simulink model "tuning_and_analysis"  (R2025b)
settings: Solver=ode45  StartTime=0.0  StopTime=0.1  RelTol=1e-6  AbsTol=1e-6
InitFcn:
  | init_pendulum
settings Model: Creator=Hp  LastModifiedBy=Hp

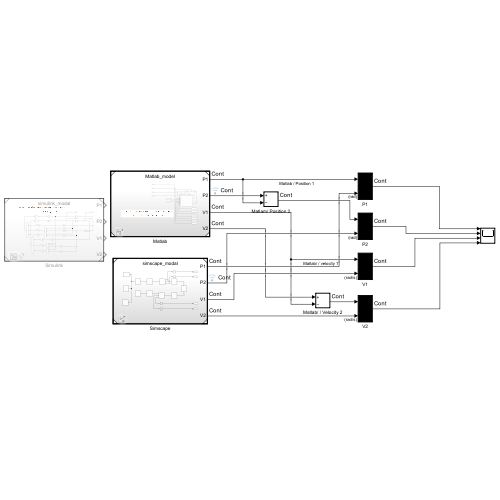
[thumbnail: Simulink's stored preview of the top-level diagram]
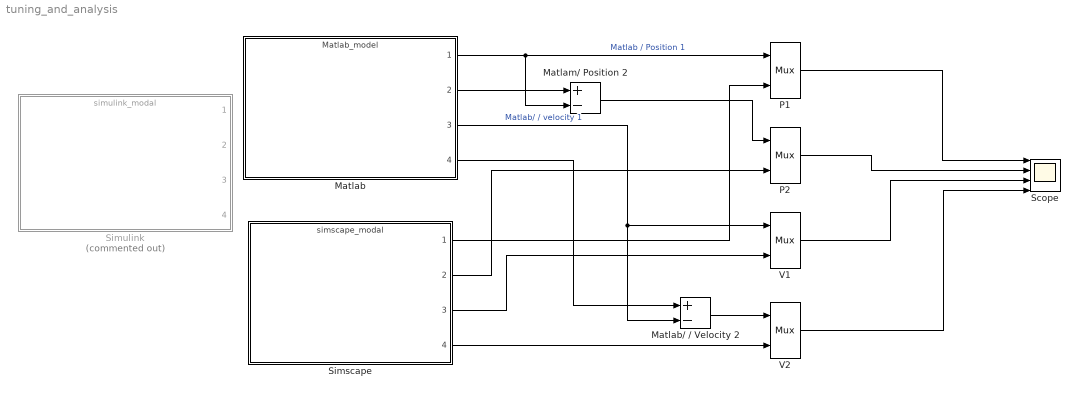
== system tuning_and_analysis ==
  Matlab : ModelReference  ModelNameDialog=Matlab_model.slx  SimulationMode=Normal  ModelReferenceVersion=1.11
  Matlab/ / Velocity 2 : Sum  Inputs=+-
  Matlam/ Position 2 : Sum  Inputs=+-
  P1 : Mux  Inputs=2
  P2 : Mux  Inputs=2
  Scope : Scope  NumInputPorts=4
      settings: ActiveDisplayYMinimum=-0.80264814806705076  ActiveDisplayYMaximum=-0.58955602599034473
  Simscape : ModelReference  ModelNameDialog=simscape_modal.slx  SimulationMode=Normal  ModelReferenceVersion=1.9
  Simulink : ModelReference  Commented=on  ModelNameDialog=simulink_modal.slx  SimulationMode=Normal  ModelReferenceVersion=1.5
  V1 : Mux  Inputs=2
  V2 : Mux  Inputs=2
  wires:
  P1/1 -> Scope/1
  P2/1 -> Scope/2
  Matlab/1 -> P1/1, Matlam/ Position 2/2  "Matlab / Position 1"
  Simscape/1 -> P1/2
  Simscape/2 -> P2/2
  Matlab/3 -> Matlab/ / Velocity 2/2, V1/1  "Matlab/ / velocity 1"
  Simscape/3 -> V1/2
  Simscape/4 -> V2/2
  Matlab/2 -> Matlam/ Position 2/1
  Matlab/ / Velocity 2/1 -> V2/1
  Matlab/4 -> Matlab/ / Velocity 2/1
  V1/1 -> Scope/3
  V2/1 -> Scope/4
  Matlam/ Position 2/1 -> P2/1
